simulink model "LMPC_1st_order_Kang_2"  (R2024b)
settings: Solver=FixedStepAuto  StartTime=0.0  StopTime=20  FixedStep=T_sample  RelTol=1e-3  EnableMultiTasking=on
undefined symbols (not defined in the file or in its folder): T_sample
settings Model: Creator=shaocan  LastModifiedBy=sk3547969879
settings SolverCC: AlgebraicLoopSolver=TrustRegion
settings DataIOCC: LimitDataPoints=on  SaveFormat=Array  ReturnWorkspaceOutputs=off
settings OptimizationCC: LifeSpan=inf
settings DebuggingCC: UnconnectedInputMsg=warning  UnconnectedOutputMsg=warning  UnconnectedLineMsg=warning  SFUnexpectedBacktrackingDiag=warning  SFNoUnconditionalDefaultTransitionDiag=warning  SFExecutionAtInitializationDiag=none  ArithmeticOperatorsInVariantConditions=warning
settings HardwareCC: ProdBitPerPointer=32  ProdBitPerSizeT=32  ProdBitPerPtrDiffT=32  ProdLargestAtomicFloat=None  ProdIntDivRoundTo=Undefined  ProdEndianess=Unspecified  ProdWordSize=32  ProdHWDeviceType=32-bit Generic
settings ModelReferenceCC: EnableRefExpFcnMdlSchedulingChecks=on  PropagateSignalLabelsOutOfModel=off
settings SFSimCC: SimUseLocalCustomCode=off  CustomCodeUndefinedFunction=UseInterfaceOnly
settings RTWCC: RTWUseLocalCustomCode=off  GPUComputeCapability=3.5
settings CodeAppCC: StateflowObjectComments=on
settings GRTTargetCC: TargetLangStandard=C89/C90 (ANSI)
settings ConfigComp: CovMetricSettings=dw  CovSaveCumulativeToWorkspaceVar=on  CovSaveSingleToWorkspaceVar=on  CovExternalEMLEnable=off  CovSFcnEnable=off

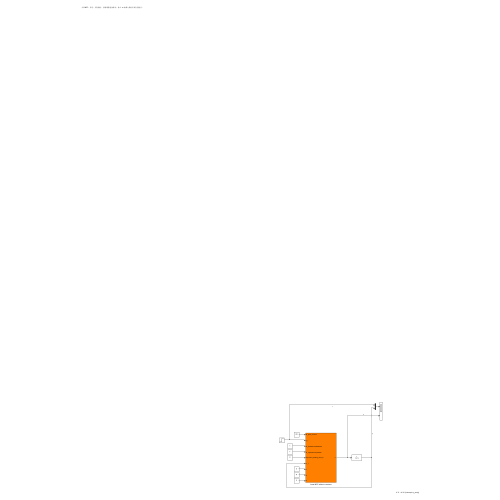
[thumbnail: Simulink's stored preview of the top-level diagram]
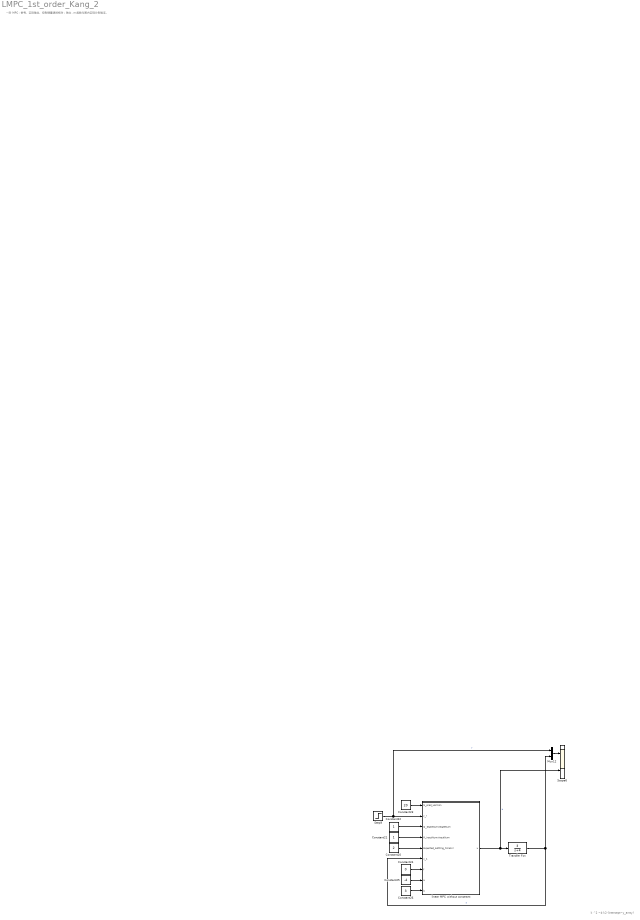
== system LMPC_1st_order_Kang_2 ==
  note: k ^2 −4⋅k2⋅(intercept−y_array)
  note: 一阶 MPC：参考、实际输出、控制增量逐拍核对；独立 .m 函数与图内实现分别验证。
  Constant20 : Constant  Value=2
  Constant21 : Constant
  Constant22 : Constant
  Constant23 : Constant  Value=20
  Constant24 : Constant  Value=0
  Constant25 : Constant  Value=-4
  Constant26 : Constant  Value=3
  Mux12 : Mux  Inputs=2
  Scope6 : Scope  NumInputPorts=2
  Step9 : Step  Time=5  Before=105  After=120  SampleTime=0
  Transfer Fcn : TransferFcn  Numerator=[3]  Denominator=[1 4]
  linear MPC without constrant : Subsystem
  wires:
  linear MPC without constrant/1(u) -> Scope6/2, Transfer Fcn/1  "u"
  Mux12/1 -> Scope6/1
  Step9/1 -> linear MPC without constrant/2(y_r), Mux12/1  "r"
  Transfer Fcn/1 -> linear MPC without constrant/6(x_1), Mux12/2  "y"
  Constant20/1 -> linear MPC without constrant/5(Expected_settling_time(s))
  Constant21/1 -> linear MPC without constrant/4(R_InputNumxInputNum)
  Constant22/1 -> linear MPC without constrant/3(Q_StateNumxStateNum)
  Constant23/1 -> linear MPC without constrant/1(N_pred_Horizon)
  Constant24/1 -> linear MPC without constrant/7(f)
  Constant25/1 -> linear MPC without constrant/8(a)
  Constant26/1 -> linear MPC without constrant/9(b)

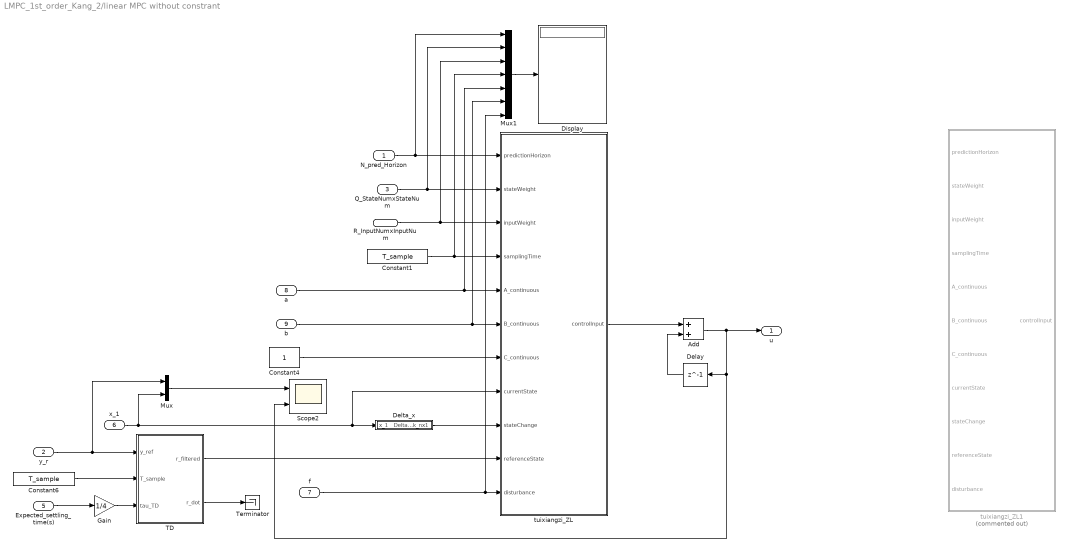
== system LMPC_1st_order_Kang_2/linear MPC without constrant ==
  N_pred_Horizon : Inport
  y_r : Inport  Port=2
  Q_StateNumxStateNum : Inport  Port=3
  R_InputNumxInputNum : Inport  Port=4
  Expected_settling_time(s) : Inport  Port=5
  x_1 : Inport  Port=6
  f : Inport  Port=7
  a : Inport  Port=8
  b : Inport  Port=9
  Add : Sum
  Constant1 : Constant  Value=T_sample
  Constant4 : Constant
  Constant6 : Constant  Value=T_sample
  Delay : Delay  DelayLength=1
  Delta_x : Subsystem
  Display : Display
  Gain : Gain  Gain=1/4
  Mux : Mux  Inputs=2
  Mux1 : Mux  Inputs=7
  Scope2 : Scope  NumInputPorts=2
  TD : Subsystem
  Terminator : Terminator
  tuixiangzi_ZL : MATLAB Function  TreatAsAtomicUnit=on
  tuixiangzi_ZL1 : MATLAB Function  Commented=on  TreatAsAtomicUnit=on
  u : Outport
  wires:
  tuixiangzi_ZL/1(controlInput) -> Add/1
  Constant1/1 -> Mux1/4, tuixiangzi_ZL/4(samplingTime)
  Add/1 -> Scope2/2, Delay/1, u/1
  Delay/1 -> Add/2
  R_InputNumxInputNum/1 -> Mux1/3, tuixiangzi_ZL/3(inputWeight)
  x_1/1 -> Mux/2, tuixiangzi_ZL/8(currentState), Delta_x/1(x_1)
  Delta_x/1(Delta_Xk_nx1) -> tuixiangzi_ZL/9(stateChange)
  f/1 -> Mux1/7, tuixiangzi_ZL/11(disturbance)
  Q_StateNumxStateNum/1 -> Mux1/2, tuixiangzi_ZL/2(stateWeight)
  N_pred_Horizon/1 -> Mux1/1, tuixiangzi_ZL/1(predictionHorizon)
  b/1 -> Mux1/6, tuixiangzi_ZL/6(B_continuous)
  Constant4/1 -> tuixiangzi_ZL/7(C_continuous)
  Constant6/1 -> TD/2(T_sample)
  TD/2(r_dot) -> Terminator/1
  Gain/1 -> TD/3(tau_TD)
  Expected_settling_time(s)/1 -> Gain/1
  y_r/1 -> Mux/1, TD/1(y_ref)
  TD/1(r_filtered) -> tuixiangzi_ZL/10(referenceState)
  Mux/1 -> Scope2/1
  a/1 -> Mux1/5, tuixiangzi_ZL/5(A_continuous)
  Mux1/1 -> Display/1

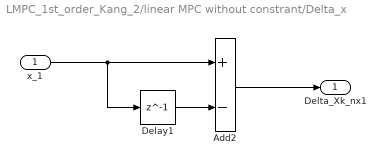
== system LMPC_1st_order_Kang_2/linear MPC without constrant/Delta_x ==
  x_1 : Inport
  Add2 : Sum  Inputs=+-
  Delay1 : Delay  DelayLength=1  InitialCondition=0
  Delta_Xk_nx1 : Outport
  wires:
  Delay1/1 -> Add2/2
  x_1/1 -> Delay1/1, Add2/1
  Add2/1 -> Delta_Xk_nx1/1

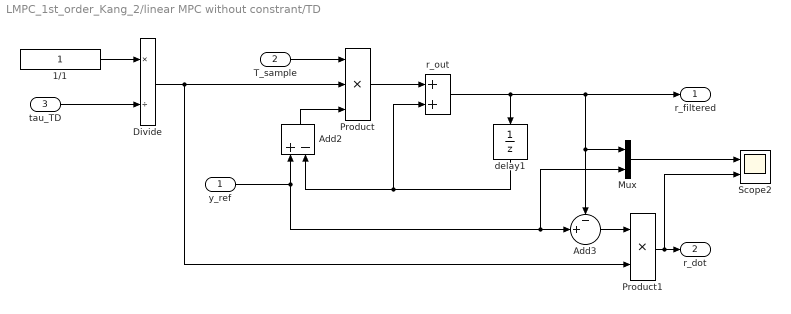
== system LMPC_1st_order_Kang_2/linear MPC without constrant/TD ==
  y_ref : Inport
  T_sample : Inport  Port=2
  tau_TD : Inport  Port=3
  1/1 : Constant
  Add2 : Sum  Inputs=+-
  Add3 : Sum  Inputs=-+|
  Divide : Product  Inputs=*/
  Mux : Mux  Inputs=2
  Product : Product  Inputs=3  RndMeth=Zero
  Product1 : Product  RndMeth=Zero
  Scope2 : Scope  NumInputPorts=2
  delay1 : UnitDelay  SampleTime=-1  HasFrameUpgradeWarning=on
  r_out : Sum
  r_filtered : Outport  VectorParamsAs1DForOutWhenUnconnected=off
  r_dot : Outport  Port=2  VectorParamsAs1DForOutWhenUnconnected=off
  wires:
  T_sample/1 -> Product/1
  Divide/1 -> Product1/2, Product/2
  Add3/1 -> Product1/1
  r_out/1 -> r_filtered/1, Mux/1, Add3/1, delay1/1
  Add2/1 -> Product/3
  Product1/1 -> Scope2/2, r_dot/1
  delay1/1 -> r_out/2, Add2/2
  y_ref/1 -> Mux/2, Add3/2, Add2/1
  Product/1 -> r_out/1
  Mux/1 -> Scope2/1
  1/1/1 -> Divide/1
  tau_TD/1 -> Divide/2

== matlab function LMPC_1st_order_Kang_2/linear MPC without constrant/tuixiangzi_ZL ==
  data: predictionHorizon input; controlInput output size=1; stateWeight input; inputWeight input; samplingTime input; A_continuous input; B_continuous input; C_continuous input; currentState input; stateChange input; referenceState input; disturbance input
function controlInput = MPC_QP(predictionHorizon, stateWeight, inputWeight, samplingTime, A_continuous, B_continuous, C_continuous, currentState, stateChange, referenceState, disturbance)
% Model Predictive Control (MPC) based on Quadratic Programming (QP)
% 
% Inputs:
% - predictionHorizon: The prediction horizon for MPC.
% - stateWeight: Weight matrix for state deviation in the cost function.
% - inputWeight: Weight matrix for control input in the cost function.
% - samplingTime: Time step for discretization.
% - A_continuous, B_continuous, C_continuous: Continuous-time system matrices.
% - currentState: The current state of the system.
% - stateChange: The difference between the current state and the previous state.
% - referenceState: The desired reference state for the system.
% - disturbance: Estimated disturbance for the system.
%
% Outputs:
% - controlInput: The computed control input based on MPC.

%%%%%%%%%%%%%%%%%%%%%%%%

% Compute the dimension of the state vector
stateDim = size(A_continuous, 1); 

% Discretize the continuous-time system matrices using Euler method
A_discrete = A_continuous .* samplingTime + eye(stateDim);
B_discrete = B_continuous .* samplingTime;
C_discrete = C_continuous .* samplingTime;

% Compute the dimension of the input vector
inputDim = size(B_discrete, 2);

% Construct the extended weight matrices for the entire prediction horizon using the Kronecker product
Q_bar = kron(eye(predictionHorizon), stateWeight);
R_bar = kron(eye(predictionHorizon), inputWeight);

% 修复：移除不必要的平方操作，直接使用权重矩阵
% 原错误代码：
% Q_bar_transpose_times_Q_bar = Q_bar' * Q_bar;
% R_bar_transpose_times_R_bar = R_bar' * R_bar;
% 修正：直接使用Q_bar和R_bar（假设它们已经是对称矩阵）

% Use repmat to create a vector by repeating the reference state for the entire prediction horizon
referenceStateAugmented = repmat(referenceState, predictionHorizon, 1);

% Initialization of matrices that will represent the prediction model over the horizon
stateMatrix = [A_discrete; zeros((predictionHorizon-1)*stateDim, stateDim)];
identityMatrix = [eye(stateDim); zeros((predictionHorizon-1)*stateDim, stateDim)];
controlMatrix = [C_discrete; zeros((predictionHorizon-1)*stateDim, inputDim)];
inputMatrix = zeros(predictionHorizon*stateDim, predictionHorizon*inputDim);

% Temporary matrices to assist in constructing the prediction model
tmpMatrix1 = A_discrete;
tmpMatrix2 = C_discrete;

% Build the prediction model matrices over the horizon
for i = 1:predictionHorizon-1
    rows = i*stateDim + (1:stateDim);
    tmpMatrix1 = A_discrete + tmpMatrix1 * A_discrete;
    stateMatrix(rows, :) = tmpMatrix1;
    identityMatrix(rows, :) = eye(stateDim);
    tmpMatrix2 = C_discrete + A_discrete * tmpMatrix2;
    controlMatrix(rows, :) = tmpMatrix2;
end

% Populate the input matrix over the horizon
inputMatrix(1:stateDim, 1:inputDim) = B_discrete;
tmpMatrix3 = B_discrete;

for i = 1:predictionHorizon-1
    rows = i*stateDim + (1:stateDim);
    tmpMatrix3 = B_discrete + A_discrete * tmpMatrix3;
    inputMatrix(rows, 1:inputDim) = tmpMatrix3;
end

% Adjust the input matrix based on the prediction horizon
for j = 1:predictionHorizon-1
    columns = j*inputDim + (1:inputDim);
    start = j*stateDim + 1;
    % 第 j 个增量对所有剩余预测步均有影响。
    stop = predictionHorizon * stateDim;
    inputMatrix(start:stop, columns) = inputMatrix(1:stop-start+1, 1:inputDim);
end

if size(controlMatrix, 2) ~= size(disturbance, 1)
    error('Dimensions of controlMatrix and disturbance do not match for multiplication');
end


% Compute the prediction error over the horizon
errorPrediction = referenceStateAugmented - stateMatrix * stateChange - identityMatrix * currentState - controlMatrix * disturbance;

% 修复：使用正确的QP公式，移除平方操作
% 原错误代码：
% controlMatrixOptimal = inputMatrix' * Q_bar_transpose_times_Q_bar * inputMatrix + R_bar_transpose_times_R_bar;
% deltaControl = controlMatrixOptimal \ inputMatrix' * Q_bar_transpose_times_Q_bar * errorPrediction;
% 修正：直接使用Q_bar和R_bar

% Compute the optimal control matrix using the pre-computed matrices
controlMatrixOptimal = inputMatrix' * Q_bar * inputMatrix + R_bar;

% Solve the quadratic program to determine the change in control input over the horizon
deltaControl = controlMatrixOptimal \ (inputMatrix' * Q_bar * errorPrediction);

% Return the first control input from the delta control sequence
controlInput = deltaControl(1:inputDim);

end

== matlab function LMPC_1st_order_Kang_2/linear MPC without constrant/tuixiangzi_ZL1 ==
  data: predictionHorizon input; controlInput output size=1; stateWeight input; inputWeight input; samplingTime input; A_continuous input; B_continuous input; C_continuous input; currentState input; stateChange input; referenceState input; disturbance input
function controlInput = MPC_QP(predictionHorizon, stateWeight, inputWeight, samplingTime, A_continuous, B_continuous, C_continuous, currentState, stateChange, referenceState, disturbance)
% Model Predictive Control (MPC) based on Quadratic Programming (QP)
% 
% Inputs:
% - predictionHorizon: The prediction horizon for MPC.
% - stateWeight: Weight matrix for state deviation in the cost function.
% - inputWeight: Weight matrix for control input in the cost function.
% - samplingTime: Time step for discretization.
% - A_continuous, B_continuous, C_continuous: Continuous-time system matrices.
% - currentState: The current state of the system.
% - stateChange: The difference between the current state and the previous state.
% - referenceState: The desired reference state for the system.
% - disturbance: Estimated disturbance for the system.
%
% Outputs:
% - controlInput: The computed control input based on MPC.

%%%%%%%%%%%%%%%%%%%%%%%%

% Compute the dimension of the state vector
stateDim = size(A_continuous, 1); 

% Discretize the continuous-time system matrices using Euler method
A_discrete = A_continuous .* samplingTime + eye(stateDim);
B_discrete = B_continuous .* samplingTime;
C_discrete = C_continuous .* samplingTime;

% Compute the dimension of the input vector
inputDim = size(B_discrete, 2);

% Construct the extended weight matrices for the entire prediction horizon using the Kronecker product
Q_bar = kron(eye(predictionHorizon), stateWeight);
R_bar = kron(eye(predictionHorizon), inputWeight);

% Pre-compute certain operations to avoid repeated calculations and enhance efficiency
Q_bar_transpose_times_Q_bar = Q_bar' * Q_bar;
R_bar_transpose_times_R_bar = R_bar' * R_bar;

% Use repmat to create a vector by repeating the reference state for the entire prediction horizon
referenceStateAugmented = repmat(referenceState, predictionHorizon, 1);

% Initialization of matrices that will represent the prediction model over the horizon
stateMatrix = [A_discrete; zeros((predictionHorizon-1)*stateDim, stateDim)];
identityMatrix = [eye(stateDim); zeros((predictionHorizon-1)*stateDim, stateDim)];
controlMatrix = [C_discrete; zeros((predictionHorizon-1)*stateDim, inputDim)];
inputMatrix = zeros(predictionHorizon*stateDim, predictionHorizon*inputDim);

% Temporary matrices to assist in constructing the prediction model
tmpMatrix1 = A_discrete;
tmpMatrix2 = C_discrete;

% Build the prediction model matrices over the horizon
for i = 1:predictionHorizon-1
    rows = i*stateDim + (1:stateDim);
    tmpMatrix1 = A_discrete + tmpMatrix1 * A_discrete;
    stateMatrix(rows, :) = tmpMatrix1;
    identityMatrix(rows, :) = eye(stateDim);
    tmpMatrix2 = C_discrete + A_discrete * tmpMatrix2;
    controlMatrix(rows, :) = tmpMatrix2;
end

% Populate the input matrix over the horizon
inputMatrix(1:stateDim, 1:inputDim) = B_discrete;
tmpMatrix3 = B_discrete;

for i = 1:predictionHorizon-1
    rows = i*stateDim + (1:stateDim);
    tmpMatrix3 = B_discrete + A_discrete * tmpMatrix3;
    inputMatrix(rows, 1:inputDim) = tmpMatrix3;
end

% Adjust the input matrix based on the prediction horizon
for j = 1:predictionHorizon-1
    columns = j*inputDim + (1:inputDim);
    start = j*stateDim + 1;
    % 第 j 个增量对所有剩余预测步均有影响。
    stop = predictionHorizon * stateDim;
    inputMatrix(start:stop, columns) = inputMatrix(1:stop-start+1, 1:inputDim);
end

if size(controlMatrix, 2) ~= size(disturbance, 1)
    error('Dimensions of controlMatrix and disturbance do not match for multiplication');
end


% Compute the prediction error over the horizon
errorPrediction = referenceStateAugmented - stateMatrix * stateChange - identityMatrix * currentState - controlMatrix * disturbance;

% Compute the optimal control matrix using the pre-computed matrices
controlMatrixOptimal = inputMatrix' * Q_bar_transpose_times_Q_bar * inputMatrix + R_bar_transpose_times_R_bar;

% Solve the quadratic program to determine the change in control input over the horizon
deltaControl = controlMatrixOptimal \ inputMatrix' * Q_bar_transpose_times_Q_bar * errorPrediction;

% Return the first control input from the delta control sequence
controlInput = deltaControl(1:inputDim);

end
